simulink model "Exp03"  (R2024b)
settings: Solver=VariableStepAuto  StartTime=0.0  StopTime=0.02  RelTol=1e-3
libraries: spsRMSLib x3, eePowerMeasurement x2, spsSeriesRLCLoadLib x2, spsVoltageMeasurementLib x2, spsACVoltageSourceLib x1, spsCurrentMeasurementLib x1, spsSeriesRLCBranchLib x1, sps_lib x1
settings Model: Creator=Siddharth  LastModifiedBy=HP

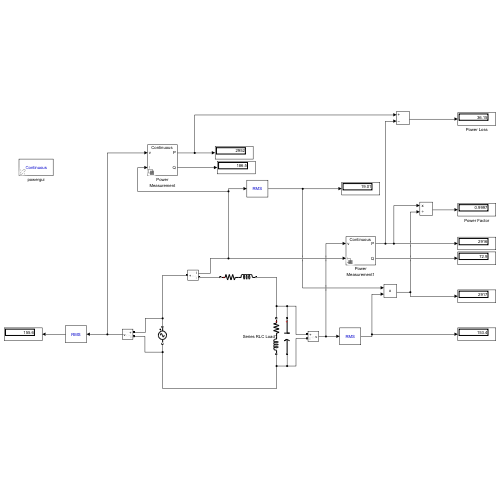
[thumbnail: Simulink's stored preview of the top-level diagram]
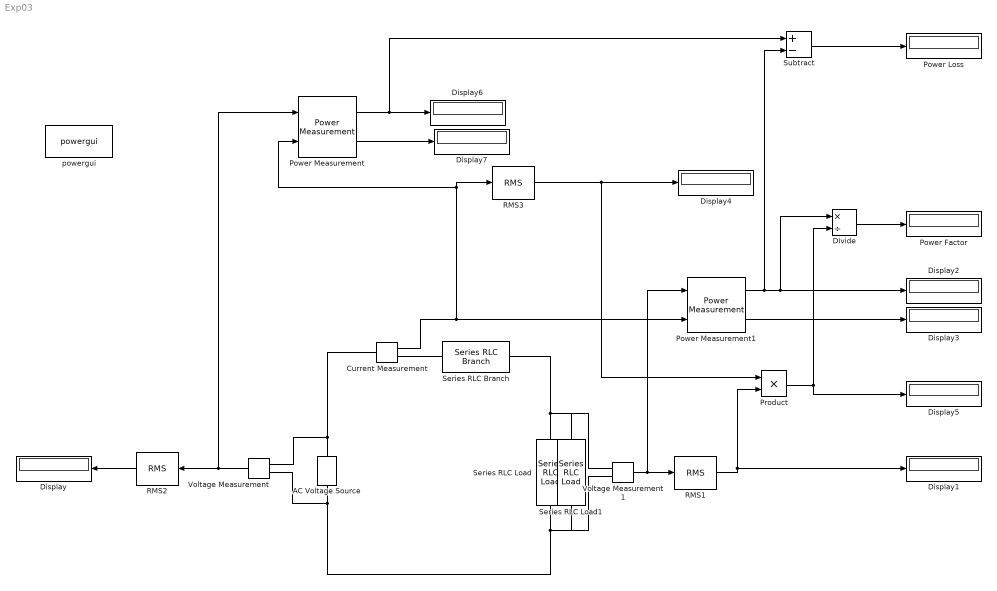
== system Exp03 ==
  AC Voltage Source : spsACVoltageSourceLib/AC Voltage Source  Amplitude=220  Phase=0  Frequency=50  SampleTime=0  Measurements=None  BusType=swing  Pref=10e3  Qref=0  Qmin=-inf  Qmax=+inf
  Current Measurement : spsCurrentMeasurementLib/Current Measurement  PhasorSimulation=off  OutputType=Complex  PSBequivalent=0
  Display{,1..7} (8 alike) : Display
  Divide : Product  Inputs=*/
  Power Measurement : eePowerMeasurement/Power Measurement  LabelModeActiveChoice=Continuous  F=50  K=[1]  Ts=0
  Power Measurement1 : eePowerMeasurement/Power Measurement  LabelModeActiveChoice=Continuous  F=50  K=[1]  Ts=0
  Power Factor : Display
  Power Loss : Display
  Product : Product
  RMS1 : spsRMSLib/RMS  TrueRMS=on  Freq=50  RMSInit=120  Ts=0
  RMS2 : spsRMSLib/RMS  TrueRMS=on  Freq=50  RMSInit=120  Ts=0
  RMS3 : spsRMSLib/RMS  TrueRMS=on  Freq=50  RMSInit=120  Ts=0
  Series RLC Branch : spsSeriesRLCBranchLib/Series RLC Branch  LConnTagsString=__new0  RConnTagsString=__new0  BranchType=RL  Resistance=0.1  Inductance=1e-3  SetiL0=off  InitialCurrent=0  Capacitance=1e-6  Setx0=off  InitialVoltage=0  Measurements=None
  Series RLC Load : spsSeriesRLCLoadLib/Series RLC Load  LConnTagsString=a  RConnTagsString=__new0  NominalVoltage=155.6  NominalFrequency=50  ActivePower=3000  InductivePower=2250  CapacitivePower=0  Setx0=off  InitialVoltage=0  SetiL0=off  InitialCurrent=0  Measurements=None  LoadType=constant Z
  Series RLC Load1 : spsSeriesRLCLoadLib/Series RLC Load  LConnTagsString=a  RConnTagsString=__new0  NominalVoltage=155.6  NominalFrequency=50  ActivePower=0  InductivePower=0  CapacitivePower=2175  Setx0=off  InitialVoltage=0  SetiL0=off  InitialCurrent=0  Measurements=None  LoadType=constant Z
  Subtract : Sum  Inputs=+-
  Voltage Measurement : spsVoltageMeasurementLib/Voltage Measurement  PhasorSimulation=off  OutputType=Complex  PSBequivalent=0
  Voltage Measurement1 : spsVoltageMeasurementLib/Voltage Measurement  PhasorSimulation=off  OutputType=Complex  PSBequivalent=0
  powergui : sps_lib/powergui  Priority=1  SimulationMode=Continuous  SampleTime=50e-6  frequency=60  Iterations=50  frequencyindice=50  Pbase=100e6  ErrMax=1e-4  UnitsV=kV  UnitsW=MW  buscounter=0  FunctionMessages=off  echomessages=off  EnableUseOfTLC=off  CurrentSourceSwitches=off  DisableSnubberDevices=off  DisableRonSwitches=off  DisableVfSwitches=off  DisplayEquations=off  AutomaticDiscreteSolvers=off  SolverType=Tustin/Backward Euler (TBE)  Interpol=off  ExternalGateDelay=off  methode=off  Ts=100  x0status=blocks  SPID=on  SwTol=0  HookPort=off  NonlinearTolerance=1e-4  nMaxIteration=100  ContinueOnMaxIteration=off  RestoreLinks=warning  ResistiveCurrentMeasurement=off  Frange=[0:2:500]  Ylog=off  Xlog=on  ShowGrid=off  save=off  variable=ZData  structure=0  ZoomFFT=off  StartTime=0.0  cycles=1  DisplayStyle=1  fundamental=60  FreqAxis=off  MaxFrequency=1000  frequencyindicesteady=1  RmsSteady=1  display=off
  wires:
  Voltage Measurement/1 -> RMS2/1, Power Measurement/1
  Voltage Measurement1/1 -> RMS1/1, Power Measurement1/1
  Power Measurement1/1 -> Subtract/2, Divide/1, Display2/1
  Power Measurement1/2 -> Display3/1
  Product/1 -> Divide/2, Display5/1
  Power Measurement/1 -> Subtract/1, Display6/1
  Power Measurement/2 -> Display7/1
  Divide/1 -> Power Factor/1
  Current Measurement/1 -> RMS3/1, Power Measurement/2, Power Measurement1/2
  Subtract/1 -> Power Loss/1
  RMS2/1 -> Display/1
  RMS3/1 -> Product/1, Display4/1
  RMS1/1 -> Product/2, Display1/1
  connections:
  AC Voltage Source/RConn1 -- Voltage Measurement/LConn1 -- Current Measurement/LConn1
  Series RLC Branch/LConn1 -- Current Measurement/RConn1
  Series RLC Branch/RConn1 -- Series RLC Load1/LConn1 -- Voltage Measurement1/LConn1 -- Series RLC Load/LConn1
  Series RLC Load/RConn1 -- Series RLC Load1/RConn1 -- Voltage Measurement1/LConn2 -- Voltage Measurement/LConn2 -- AC Voltage Source/LConn1
